simulink model "PV_GFL_864_Average_SM_R1"  (R2026a)
settings: Solver=ode23t  StopTime=0.20  MaxStep=1e-5
InitFcn:
  | run(fullfile(fileparts(get_param(bdroot,'FileName')),'..','scripts','init_pv_gfl_864_average_sm.m'));
undefined symbols (not defined in the file): Control, DiscIntNeverNeededParam, ee, GridTransformer, S1, SM, Ts
libraries: ee_lib x18, nesl_utility x16, fl_lib x10, simulink x1, eeSmAC1C x1
Description:
  | B2 readable SRF-PLL, dq measurement, and P/Q estimation on the validated B1 switching plant.
settings Model: Creator=fakebob2004  LastModifiedBy=fakebob2004

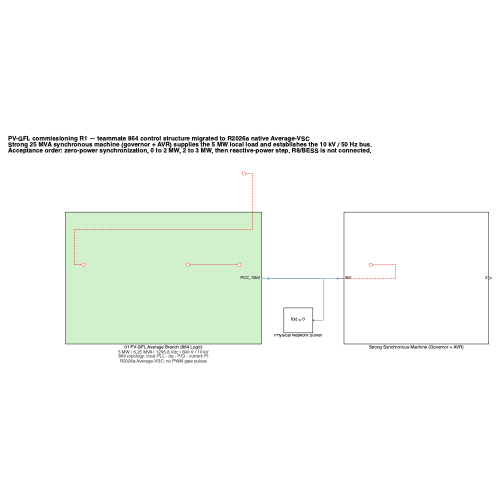
[thumbnail: Simulink's stored preview of the top-level diagram]
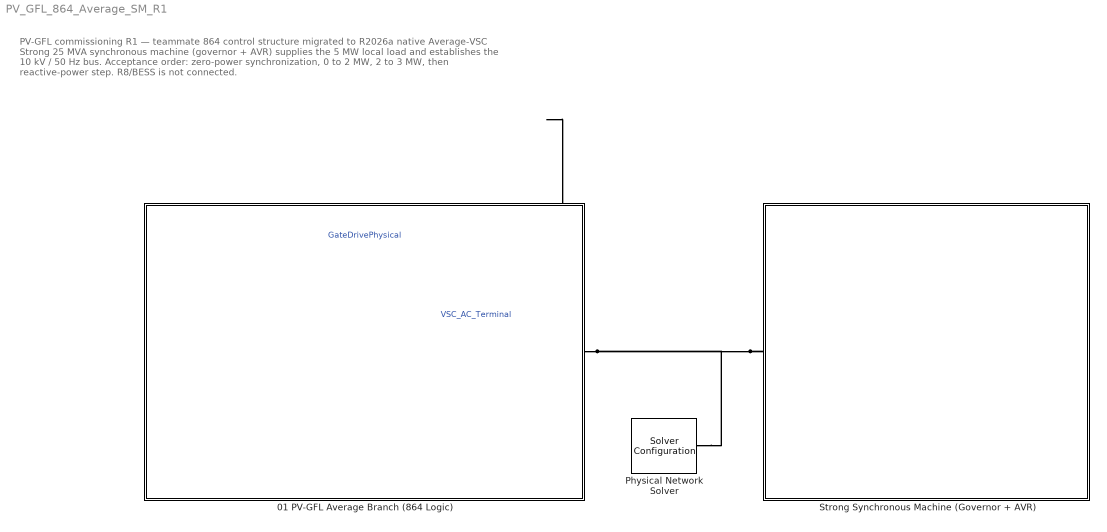
== system PV_GFL_864_Average_SM_R1 ==
  note: PV-GFL commissioning R1 — teammate 864 control structure migrated to R2026a native Average-VSC
      | Strong 25 MVA synchronous machine (governor + AVR) supplies the 5 MW local load and establishes the 10 kV / 50 Hz bus.
      | Acceptance order: zero-power synchronization, 0 to 2 MW, 2 to 3 MW, then reactive-power step. R8/BESS is not connected.
  01 PV-GFL Average Branch (864 Logic) : Subsystem
      settings: AttributesFormatString=|
      | 5 MW / 6.25 MVA | 1295.8 Vdc | 690 V / 10 kV
      | 864 topology: local PLL - dq - P/Q - current PI
      | R2026a Average-VSC; no PWM gate pulses
  Physical Network Solver : nesl_utility/Solver Configuration  PhysicalDomain=network_engine_domain  SubClassName=solver  LeftPortType=input  RightPortType=generic  Tones=[]  Harmonics=[]  SimulateNoise=off  Profile=off  UseLocalSampling=off  EnableSwitchedLinearOptims=on  FrequencyDomain=off  UseCCode=off  RelTol=0.001  AbsTol=0.001  MinStep=1e-09  ToWorkspace=off  RevertToSquareIcSolve=off  NumHomotopyIterations=100  PhasorMode=off  PhasorModeNumHarmonics=1  ConsistencySolver=NEWTON_XTOL_AFTER_FTOL  CanonicalOrdering=CANONICAL  OptimizeIntermediates=OPTIMIZED  IndexReductionMethod=DerivativeReplacement  DoDC=off  ResidualTolerance=1e-09  ConsistencyTolSource=GLOBAL  ConsistencyAbsTol=0.001  ConsistencyRelTol=0.001  ConsistencyTolFactor=0.001  UseLocalSolver=off  LocalSolverChoice=NE_BACKWARD_EULER_ADVANCER  ResolveIndetEquations=on  FunctionEvalNumThread=1  LocalSolverSampleTime=0.001  DoFixedCost=off  MaxNonlinIter=3  MaxModeIter=2  ComputeImpulses=off  ImpulseIterations=2  LinearAlgebra=auto  LinearAlgebraNumThread=0  EquationFormulation=NE_TIME_EF  DelaysMemoryBudget=1024  AutomaticFiltering=on  FilteringTimeConstant=0.001  PartitionStorageMethod=AS_NEEDED  PartitionMemoryBudget=1024  PartitionMethod=ROBUST  MultibodyUseLocalSolver=off  MultibodyLocalSolverChoice=ODE1  MultibodyLocalSolverSampleTime=0.001
  Strong Synchronous Machine (Governor + AVR) : Subsystem  VariantControl=SynchronousMachine
  connections:
  ?  "VSC_AC_Terminal"
  ?  "GateDrivePhysical"
  Strong Synchronous Machine (Governor + AVR)/RConn1 -- 01 PV-GFL Average Branch (864 Logic)/RConn1 -- Physical Network Solver/RConn1

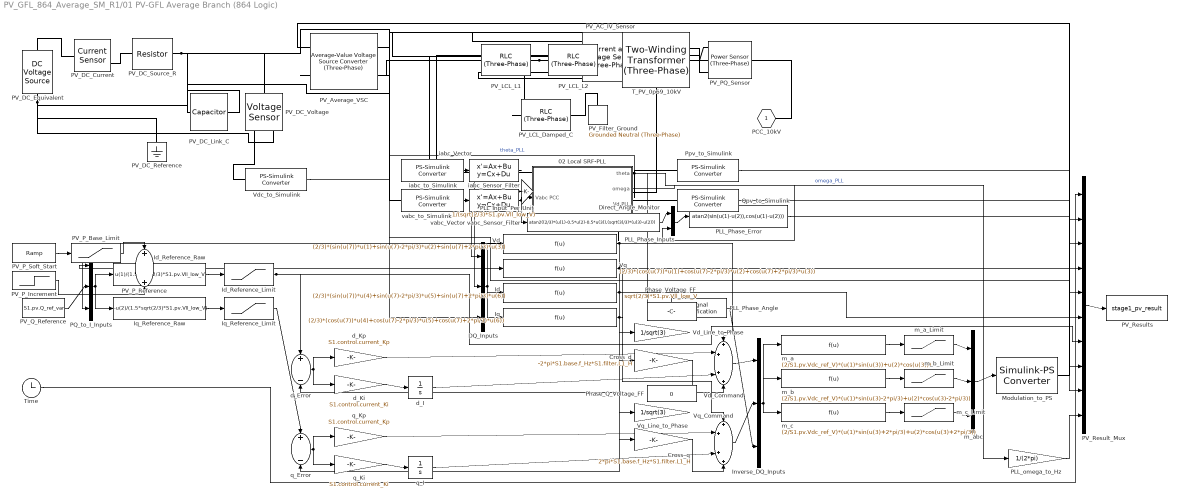
== system PV_GFL_864_Average_SM_R1/01 PV-GFL Average Branch (864 Logic) ==
  02 Local SRF-PLL : Subsystem
  Cross_d : Gain  Gain=-2*pi*S1.base.f_Hz*S1.filter.L1_H
  Cross_q : Gain  Gain=2*pi*S1.base.f_Hz*S1.filter.L1_H
  DQ_Inputs : Mux  Inputs=3
  Direct_Angle_Monitor : Fcn  Expr=atan2((2/3)*(u(1)-0.5*u(2)-0.5*u(3)),(sqrt(3)/3)*(u(3)-u(2)))
  Id : Fcn  Expr=(2/3)*(sin(u(7))*u(4)+sin(u(7)-2*pi/3)*u(5)+sin(u(7)+2*pi/3)*u(6))
  Id_Reference_Limit : Saturate  UpperLimit=S1.control.Ilimit_A  LowerLimit=-S1.control.Ilimit_A
  Id_Reference_Raw : Fcn  Expr=u(1)/(1.5*sqrt(2/3)*S1.pv.Vll_low_V)
  Inverse_DQ_Inputs : Mux  Inputs=3
  Iq : Fcn  Expr=(2/3)*(cos(u(7))*u(4)+cos(u(7)-2*pi/3)*u(5)+cos(u(7)+2*pi/3)*u(6))
  Iq_Reference_Limit : Saturate  UpperLimit=S1.control.Ilimit_A  LowerLimit=-S1.control.Ilimit_A
  Iq_Reference_Raw : Fcn  Expr=-u(2)/(1.5*sqrt(2/3)*S1.pv.Vll_low_V)
  Modulation_to_PS : nesl_utility/Simulink-PS Converter  PhysicalDomain=network_engine_domain  SubClassName=ps_input  LeftPortType=input  RightPortType=output  PseudoPeriodic=off  Frequencies=[]  NoiseDistribution=none  NoiseParameters=[]  Unit=1  AffineConversion=off  FilteringAndDerivatives=zero  SimscapeFilterOrder=1  InputFilterTimeConstant=0.001  UdotUserProvided=0
  PLL_Input_Per_Unit : Gain  Gain=1/(sqrt(2/3)*S1.pv.Vll_low_V)
  PLL_Phase_Angle : SignalSpecification
  PLL_Phase_Error : Fcn  Expr=atan2(sin(u(1)-u(2)),cos(u(1)-u(2)))
  PLL_Phase_Inputs : Mux  Inputs=2
  PLL_omega_to_Hz : Gain  Gain=1/(2*pi)
  PQ_to_I_Inputs : Mux  Inputs=3
  PV_AC_IV_Sensor : ee_lib/Sensors & Transducers/Current and Voltage Sensor (Three-Phase)  port_option=ee.enum.threePhasePort.composite  vMeasurementType=ee.enum.vmeasurement.ll  outputUnit=ee.enum.unit.si  SRated=100e6 A*V  VRated=24e3 V  I_specify=off  I_priority=None  I=[0, 0, 0] A  I_nominal_specify=off  I_nominal_value=1  I_nominal_unit=A  V_specify=off  V_priority=None  V=[0, 0, 0] V  V_nominal_specify=off  V_nominal_value=1  V_nominal_unit=V
  PV_Average_VSC : ee_lib/Semiconductors & Converters/Converters/Average-Value Voltage Source Converter (Three-Phase)  port_option=ee.enum.threePhasePort.composite  enable_block_pulses_input=false  krec=0.001 Ohm  frequency_option=ee.enum.converters.frequency.variable  input_option=ee.enum.converters.inputOption.ModWave  FRated=S1.base.f_Hz Hz  losses_parameterization=ee.enum.converters.losses.fixed  Pfixed=1 W  ks=0.01  kc1=1.7 V  kc2=0.01 Ohm  Ploss_vect=[100, 800, 1870, 3250, 4900] W  Irms_vect=[10, 100, 200, 300, 400] A  Vdc_nom=300 V  thermal_mass=30000 J/K  temperature_specify=off  temperature_priority=High  temperature=298.15 K  temperature_nominal_specify=off  temperature_nominal_value=1  temperature_nominal_unit=K
  PV_DC_Current : fl_lib/Electrical/Electrical Sensors/Current Sensor
  PV_DC_Equivalent : fl_lib/Electrical/Electrical Sources/DC Voltage Source  v0=S1.pv.Vdc_ref_V V
  PV_DC_Link_C : fl_lib/Electrical/Electrical Elements/Capacitor  c=S1.pv.Cdc_F F  r=1e-6 Ohm  g=0 1/Ohm  i_specify=off  i_priority=None  i=0 A  i_nominal_specify=off  i_nominal_value=1  i_nominal_unit=A  v_specify=off  v_priority=None  v=0 V  v_nominal_specify=off  v_nominal_value=1  v_nominal_unit=V  vc_specify=on  vc_priority=High  vc=S1.pv.Vdc_ref_V V  vc_nominal_specify=off  vc_nominal_value=1  vc_nominal_unit=V
  PV_DC_Reference : fl_lib/Electrical/Electrical Elements/Electrical Reference
  PV_DC_Source_R : fl_lib/Electrical/Electrical Elements/Resistor  R=S1.pv.dc_source_R_ohm Ohm  i_specify=off  i_priority=None  i=0 A  i_nominal_specify=off  i_nominal_value=1  i_nominal_unit=A  v_specify=off  v_priority=None  v=0 V  v_nominal_specify=off  v_nominal_value=1  v_nominal_unit=V
  PV_DC_Voltage : fl_lib/Electrical/Electrical Sensors/Voltage Sensor
  PV_Filter_Ground : ee_lib/Connectors & References/Grounded Neutral (Three-Phase)  port_option=ee.enum.threePhasePort.composite
  PV_LCL_Damped_C : ee_lib/Passive/RLC Assemblies/RLC (Three-Phase)  port_option=ee.enum.threePhasePort.composite  component_structure=ee.enum.rlc.structure.SeriesRC  R=S1.filter.Rd_ohm Ohm  L=1e-3 H  C=S1.filter.C_F F  R_parasitic=0 Ohm  G_parasitic=0 1/Ohm  IL_specify=off  IL_priority=High  IL=[0, 0, 0] A  IL_nominal_specify=off  IL_nominal_value=1  IL_nominal_unit=A  VC_specify=off  VC_priority=High  VC=[0, 0, 0] V  VC_nominal_specify=off  VC_nominal_value=1  VC_nominal_unit=V
  PV_LCL_L1 : ee_lib/Passive/RLC Assemblies/RLC (Three-Phase)  port_option=ee.enum.threePhasePort.composite  component_structure=ee.enum.rlc.structure.SeriesRL  R=S1.filter.R1_ohm Ohm  L=S1.filter.L1_H H  C=1e-6 F  R_parasitic=0 Ohm  G_parasitic=0 1/Ohm  IL_specify=off  IL_priority=High  IL=[0, 0, 0] A  IL_nominal_specify=off  IL_nominal_value=1  IL_nominal_unit=A  VC_specify=off  VC_priority=High  VC=[0, 0, 0] V  VC_nominal_specify=off  VC_nominal_value=1  VC_nominal_unit=V
  PV_LCL_L2 : ee_lib/Passive/RLC Assemblies/RLC (Three-Phase)  port_option=ee.enum.threePhasePort.composite  component_structure=ee.enum.rlc.structure.SeriesRL  R=S1.filter.R2_ohm Ohm  L=S1.filter.L2_H H  C=1e-6 F  R_parasitic=0 Ohm  G_parasitic=0 1/Ohm  IL_specify=off  IL_priority=High  IL=[0, 0, 0] A  IL_nominal_specify=off  IL_nominal_value=1  IL_nominal_unit=A  VC_specify=off  VC_priority=High  VC=[0, 0, 0] V  VC_nominal_specify=off  VC_nominal_value=1  VC_nominal_unit=V
  PV_PQ_Sensor : ee_lib/Sensors & Transducers/Power Sensor (Three-Phase)  port_option=ee.enum.threePhasePort.composite  load_type=ee.enum.passive.type_balanced.balanced  f0=60 Hz
  PV_P_Base_Limit : Saturate  UpperLimit=S1.pv.P_initial_W  LowerLimit=0
  PV_P_Increment : Step  Time=S1.pv.P_step_time_s  FinalValue=S1.pv.P_final_W-S1.pv.P_initial_W  SampleTime=0
  PV_P_Reference : Sum
  PV_P_Soft_Start : simulink/Sources/Ramp  slope=S1.pv.P_ramp_W_per_s  start=0  InitialOutput=0
  PV_Q_Reference : Constant  Value=S1.pv.Q_ref_var
  PV_Result_Mux : Mux  Inputs=10
  PV_Results : ToWorkspace  VariableName=stage1_pv_result  SampleTime=-1
  Phase_Q_Voltage_FF : Constant  Value=0
  Phase_Voltage_FF : Constant  Value=sqrt(2/3)*S1.pv.Vll_low_V
  Ppv_to_Simulink : nesl_utility/PS-Simulink Converter  PhysicalDomain=network_engine_domain  SubClassName=ps_output  LeftPortType=input  RightPortType=output  PseudoPeriodic=off  Frequencies=[]  VectorFormat=inherit  Unit=W  AffineConversion=off
  Qpv_to_Simulink : nesl_utility/PS-Simulink Converter  PhysicalDomain=network_engine_domain  SubClassName=ps_output  LeftPortType=input  RightPortType=output  PseudoPeriodic=off  Frequencies=[]  VectorFormat=inherit  Unit=W  AffineConversion=off
  T_PV_0p69_10kV : ee_lib/Passive/Transformers/Two-Winding Transformer (Three-Phase)  SRated=S1.transformer.S_VA A*V  FRated=S1.base.f_Hz Hz  Winding1Connection=ee.enum.windingconnection.delta1  VRated1=S1.pv.Vll_low_V V  Winding2Connection=ee.enum.windingconnection.Yg  VRated2=S1.pv.Vll_high_V V  CoreType=ee.enum.coretype.threelimb  pu_Rw1=S1.transformer.R_pu/2  pu_Rw2=S1.transformer.R_pu/2  leakage_reactance_option=ee.enum.transformer_leakage.include  pu_Xl1=S1.transformer.X_pu/2  pu_Xl2=S1.transformer.X_pu/2  magnetizing_resistance_option=ee.enum.transformer_magnetizingResistance.exclude  pu_Rm=500  magnetizing_reactance_option=ee.enum.transformer_magnetizingReactance.exclude  saturation_option=ee.enum.transformer_saturation.exclude  pu_Xm=500  current_data=[0, .002, 1, 2]  magnetic_flux_data=[0, 1.2, 1.5, 1.51]  pu_X0=0.5  i1_specify=off  i1_priority=None  i1=[0, 0, 0] A  i1_nominal_specify=off  i1_nominal_value=1  i1_nominal_unit=A  i2_specify=off  i2_priority=None  i2=[0, 0, 0] A  i2_nominal_specify=off  i2_nominal_value=1  i2_nominal_unit=A  phi_specify=off  phi_priority=None  phi=[0, 0, 0]  phi_nominal_specify=off  phi_nominal_value=1  phi_nominal_unit=1
  Time : Clock
  Vd : Fcn  Expr=(2/3)*(sin(u(7))*u(1)+sin(u(7)-2*pi/3)*u(2)+sin(u(7)+2*pi/3)*u(3))
  Vd_Command : Sum  Inputs=++++
  Vd_Line_to_Phase : Gain  Gain=1/sqrt(3)
  Vdc_to_Simulink : nesl_utility/PS-Simulink Converter  PhysicalDomain=network_engine_domain  SubClassName=ps_output  LeftPortType=input  RightPortType=output  PseudoPeriodic=off  Frequencies=[]  VectorFormat=inherit  Unit=V  AffineConversion=off
  Vq : Fcn  Expr=(2/3)*(cos(u(7))*u(1)+cos(u(7)-2*pi/3)*u(2)+cos(u(7)+2*pi/3)*u(3))
  Vq_Command : Sum  Inputs=++++
  Vq_Line_to_Phase : Gain  Gain=1/sqrt(3)
  d_Error : Sum  Inputs=+-
  d_I : Integrator
  d_Ki : Gain  Gain=S1.control.current_Ki
  d_Kp : Gain  Gain=S1.control.current_Kp
  iabc_Sensor_Filter : StateSpace  A=-eye(3)/S1.control.sensor_filter_s  B=eye(3)/S1.control.sensor_filter_s  C=eye(3)  D=zeros(3)  InitialCondition=zeros(3,1)
  iabc_Vector : Reshape
  iabc_to_Simulink : nesl_utility/PS-Simulink Converter  PhysicalDomain=network_engine_domain  SubClassName=ps_output  LeftPortType=input  RightPortType=output  PseudoPeriodic=off  Frequencies=[]  VectorFormat=inherit  Unit=A  AffineConversion=off
  m_a : Fcn  Expr=(2/S1.pv.Vdc_ref_V)*(u(1)*sin(u(3))+u(2)*cos(u(3)))
  m_a_Limit : Saturate  UpperLimit=S1.pv.modulation_max  LowerLimit=-S1.pv.modulation_max
  m_abc : Mux  Inputs=3
  m_b : Fcn  Expr=(2/S1.pv.Vdc_ref_V)*(u(1)*sin(u(3)-2*pi/3)+u(2)*cos(u(3)-2*pi/3))
  m_b_Limit : Saturate  UpperLimit=S1.pv.modulation_max  LowerLimit=-S1.pv.modulation_max
  m_c : Fcn  Expr=(2/S1.pv.Vdc_ref_V)*(u(1)*sin(u(3)+2*pi/3)+u(2)*cos(u(3)+2*pi/3))
  m_c_Limit : Saturate  UpperLimit=S1.pv.modulation_max  LowerLimit=-S1.pv.modulation_max
  q_Error : Sum  Inputs=+-
  q_I : Integrator
  q_Ki : Gain  Gain=S1.control.current_Ki
  q_Kp : Gain  Gain=S1.control.current_Kp
  vabc_Sensor_Filter : StateSpace  A=-eye(3)/S1.control.sensor_filter_s  B=eye(3)/S1.control.sensor_filter_s  C=eye(3)  D=zeros(3)  InitialCondition=sqrt(2/3)*S1.pv.Vll_low_V*[sin(pi/6);sin(pi/6-2*pi/3);sin(pi/6+2*pi/3)]
  vabc_Vector : Reshape
  vabc_to_Simulink : nesl_utility/PS-Simulink Converter  PhysicalDomain=network_engine_domain  SubClassName=ps_output  LeftPortType=input  RightPortType=output  PseudoPeriodic=off  Frequencies=[]  VectorFormat=inherit  Unit=V  AffineConversion=off
  PCC_10kV : PMIOPort  Side=Right  ConnectionType=Connection: foundation.electrical.three_phase
  wires:
  PV_Result_Mux/1 -> PV_Results/1
  Vdc_to_Simulink/1 -> PV_Result_Mux/9
  PLL_Phase_Error/1 -> PV_Result_Mux/5
  Qpv_to_Simulink/1 -> PV_Result_Mux/3
  Ppv_to_Simulink/1 -> PV_Result_Mux/2
  Time/1 -> PV_Result_Mux/1
  m_abc/1 -> Modulation_to_PS/1
  m_c_Limit/1 -> m_abc/3
  m_b_Limit/1 -> m_abc/2
  m_a_Limit/1 -> m_abc/1
  m_c/1 -> m_c_Limit/1
  m_b/1 -> m_b_Limit/1
  m_a/1 -> m_a_Limit/1
  Inverse_DQ_Inputs/1 -> m_c/1, m_b/1, m_a/1
  PLL_Phase_Angle/1 -> Inverse_DQ_Inputs/3
  Vq_Command/1 -> Inverse_DQ_Inputs/2
  Vd_Command/1 -> Inverse_DQ_Inputs/1
  Cross_q/1 -> Vq_Command/4
  q_I/1 -> Vq_Command/3
  q_Kp/1 -> Vq_Command/2
  Cross_d/1 -> Vd_Command/4
  d_I/1 -> Vd_Command/3
  d_Kp/1 -> Vd_Command/2
  Vq/1 -> Vq_Line_to_Phase/1, Vq_Command/1
  Iq/1 -> PV_Result_Mux/7, Cross_d/1, q_Error/2
  Iq_Reference_Limit/1 -> q_Error/1
  Id/1 -> PV_Result_Mux/6, Cross_q/1, d_Error/2
  Id_Reference_Limit/1 -> PV_Result_Mux/8, d_Error/1
  q_Ki/1 -> q_I/1
  q_Error/1 -> q_Ki/1, q_Kp/1
  d_Ki/1 -> d_I/1
  d_Error/1 -> d_Ki/1, d_Kp/1
  Iq_Reference_Raw/1 -> Iq_Reference_Limit/1
  Id_Reference_Raw/1 -> Id_Reference_Limit/1
  PQ_to_I_Inputs/1 -> Iq_Reference_Raw/1, Id_Reference_Raw/1
  Vd/1 -> Vd_Line_to_Phase/1, PQ_to_I_Inputs/3, Vd_Command/1
  PV_Q_Reference/1 -> PQ_to_I_Inputs/2
  PV_P_Reference/1 -> PV_Result_Mux/4, PQ_to_I_Inputs/1
  PV_P_Increment/1 -> PV_P_Reference/2
  PV_P_Base_Limit/1 -> PV_P_Reference/1
  PV_P_Soft_Start/1 -> PV_P_Base_Limit/1
  DQ_Inputs/1 -> Iq/1, Id/1, Vq/1, Vd/1
  iabc_Sensor_Filter/1 -> DQ_Inputs/2
  PLL_Phase_Inputs/1 -> PLL_Phase_Error/1
  Direct_Angle_Monitor/1 -> PLL_Phase_Inputs/1
  vabc_Sensor_Filter/1 -> DQ_Inputs/1, Direct_Angle_Monitor/1, PLL_Input_Per_Unit/1, 02 Local SRF-PLL/1(Vabc PCC)
  vabc_Vector/1 -> vabc_Sensor_Filter/1
  iabc_Vector/1 -> iabc_Sensor_Filter/1
  vabc_to_Simulink/1 -> vabc_Vector/1
  iabc_to_Simulink/1 -> iabc_Vector/1
  02 Local SRF-PLL/1(theta) -> PLL_Phase_Inputs/2, DQ_Inputs/3, PLL_Phase_Angle/1  "theta_PLL"
  02 Local SRF-PLL/2(omega) -> PLL_omega_to_Hz/1  "omega_PLL"
  PLL_omega_to_Hz/1 -> PV_Result_Mux/10
  connections:
  Modulation_to_PS/RConn1 -- PV_Average_VSC/LConn1
  PV_DC_Voltage/RConn1 -- Vdc_to_Simulink/LConn1
  PV_PQ_Sensor/LConn3 -- Qpv_to_Simulink/LConn1
  PV_PQ_Sensor/LConn2 -- Ppv_to_Simulink/LConn1
  PV_AC_IV_Sensor/RConn1 -- vabc_to_Simulink/LConn1
  PV_AC_IV_Sensor/RConn2 -- iabc_to_Simulink/LConn1
  PV_PQ_Sensor/RConn1 -- PCC_10kV/RConn1
  T_PV_0p69_10kV/RConn1 -- PV_PQ_Sensor/LConn1
  PV_LCL_Damped_C/RConn1 -- PV_Filter_Ground/LConn1
  PV_LCL_Damped_C/LConn1 -- PV_LCL_L1/RConn1 -- PV_LCL_L2/LConn1
  PV_DC_Reference/LConn1 -- PV_DC_Voltage/RConn2 -- PV_DC_Link_C/RConn1 -- PV_DC_Equivalent/RConn1 -- PV_Average_VSC/RConn2
  PV_DC_Voltage/LConn1 -- PV_DC_Link_C/LConn1 -- PV_DC_Source_R/RConn1 -- PV_Average_VSC/RConn1
  PV_DC_Current/RConn2 -- PV_DC_Source_R/LConn1
  PV_DC_Equivalent/LConn1 -- PV_DC_Current/LConn1
  PV_Average_VSC/LConn2 -- PV_LCL_L1/LConn1
  PV_LCL_L2/RConn1 -- PV_AC_IV_Sensor/LConn1
  PV_AC_IV_Sensor/RConn3 -- T_PV_0p69_10kV/LConn1

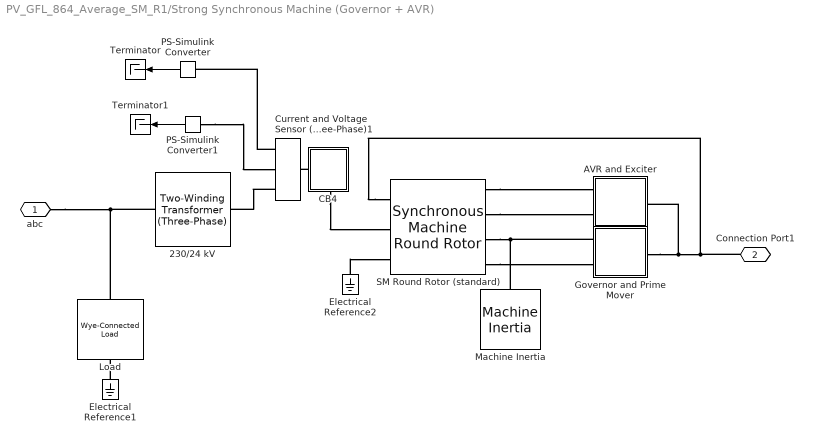
== system PV_GFL_864_Average_SM_R1/Strong Synchronous Machine (Governor + AVR) ==
  " Load" : ee_lib/Passive/RLC Assemblies/Wye-Connected Load  port_option=ee.enum.threePhasePort.composite  parameterization=ee.enum.rlc.parameterization.ratedpower  component_structure=ee.enum.rlc.structure.R  component_structure_PQ=ee.enum.rlc.structure.ParallelRL  R=1 Ohm  L=1e-3 H  C=1e-6 F  VRated=Grid.voltage V  FRated=Grid.frequency Hz  P=SM.P_load W  Qpos=SM.Q_load A*V  Qneg=-1e2 A*V  R_parasitic=0 Ohm  G_parasitic=0 1/Ohm  R_parasitic_PQ=0 Ohm  G_parasitic_PQ=0 1/Ohm  Vmag0=4.16e3 V  Vang0=0 deg  Freq0=60 Hz  IL_specify=off  IL_priority=High  IL=[0, 0, 0] A  IL_nominal_specify=off  IL_nominal_value=1  IL_nominal_unit=A  VC_specify=off  VC_priority=High  VC=[0, 0, 0] V  VC_nominal_specify=off  VC_nominal_value=1  VC_nominal_unit=V
  230/24 kV : ee_lib/Passive/Transformers/Two-Winding Transformer (Three-Phase)  SRated=SM.MVA V*A  FRated=Grid.frequency Hz  Winding1Connection=ee.enum.windingconnection.delta1  VRated1=Grid.voltage V  Winding2Connection=ee.enum.windingconnection.delta11  VRated2=SM.Voltage V  CoreType=ee.enum.coretype.fivelimb  pu_Rw1=GridTransformer.winding_resistance/2  pu_Rw2=GridTransformer.winding_resistance/2  leakage_reactance_option=ee.enum.transformer_leakage.include  pu_Xl1=GridTransformer.winding_lekage_reactance/2  pu_Xl2=GridTransformer.winding_lekage_reactance/2  magnetizing_resistance_option=ee.enum.transformer_magnetizingResistance.exclude  pu_Rm=500  magnetizing_reactance_option=ee.enum.transformer_magnetizingReactance.include  saturation_option=ee.enum.transformer_saturation.exclude  pu_Xm=500  current_data=[0, .002, 1, 2]  magnetic_flux_data=[0, 1.2, 1.5, 1.51]  pu_X0=0.0586/2  i1_specify=off  i1_priority=None  i1=[ 0 0 0 ] A  i1_nominal_specify=off  i1_nominal_value=1  i1_nominal_unit=A  i2_specify=off  i2_priority=None  i2=[ 0 0 0 ] A  i2_nominal_specify=off  i2_nominal_value=1  i2_nominal_unit=A  phi_specify=off  phi_priority=None  phi=[ 0 0 0 ]  phi_nominal_specify=off  phi_nominal_value=1  phi_nominal_unit=1
  AVR and Exciter : Subsystem
  CB4 : Subsystem
      settings: PortSchema="{\"entries\":[{\"content\":{\"sides\":[{\"content\":{\"connectorIds\":[\"LConn1\"]},\"type\":\"ConnectorPlacement.EquallySpacedRectSide\",\"uuid\":\"24022911-97b6-486c-a625-f0780a134feb\"},{\"content\":{\"connectorIds\":[],\"side\":\"RIGHT\"},\"type\":\"ConnectorPlacement.EquallySpacedRectSide\",\"uuid\":\"1242aa8b-343b-4af2-8b96-dfa58505a53d\"},{\"content\":{\"connectorIds\":[],\"side\":\"TOP\"},\"type\":\"ConnectorPlacement.EquallySpacedRectSide\",\"uuid\":\"e73be2e9-5300-480f-914f-665ff518f6ad\"},{\"content\":{\"connectorIds\":[\"RConn1\"],\"side\":\"BOTTOM\"},\"type\":\"ConnectorPlacement.EquallySpacedRectSide\",\"uuid\":\"6525202c-c4e7-4c96-9421-427b801d0594\"}]},\"type\":\"ConnectorPlacement.EquallySpacedConnector\",\"uuid\":\"b455682c-e951-4ef6-bff8-cd3f50b315f1\"}],\"packageUris\":[\"http://schema.mathworks.com/mf0/Connector/R2020b\"],\"version\":\"1.0\"}"
      mask Display: image('$imagefile'); % Use "Edit Image" on toolstrip to change.
  Current and Voltage Sensor (Three-Phase)1 : ee_lib/Sensors & Transducers/Current and Voltage Sensor (Three-Phase)  port_option=ee.enum.threePhasePort.composite  vMeasurementType=ee.enum.vmeasurement.ll  outputUnit=ee.enum.unit.pu  SRated=100e6 A*V  VRated=4.16e3 V  I_specify=off  I_priority=None  I=[0, 0, 0] A  I_nominal_specify=off  I_nominal_value=1  I_nominal_unit=A  V_specify=off  V_priority=None  V=[0, 0, 0] V  V_nominal_specify=off  V_nominal_value=1  V_nominal_unit=V
  Electrical Reference1 : fl_lib/Electrical/Electrical Elements/Electrical Reference
  Electrical Reference2 : fl_lib/Electrical/Electrical Elements/Electrical Reference
  "Governor and Prime Mover " : Subsystem  mask(Governor and Prime Mover){pu_speed_reference=SM.speed_reference, droop_percentage=SM.droop_p, pu_load_reference_setpoint=SM.load_reference_set_point, T_G=SM.governor_time_constant, T_CH=SM.time_constsnt_steamchest, base_torque=SM.Base_Torque_SM, pu_torque0=SM.initial_torque}
      mask prompts: pu_speed_reference "Speed reference, (pu)"; droop_percentage "Percentage droop, (%)"; pu_load_reference_setpoint "Load reference setpoint, (pu)"; T_G "Time constant of governor, (s)"; T_CH "Time constant of main inlet volumes and steam chest, (s)"; base_torque "Base torque, (N*m)"; pu_torque0 "Initial torque, (pu)"
      mask help:
      | Implements a synchronous machine governor and prime mover. The prime mover is a non-reheat steam turbine.
      |
      | The input to the block is a per-unit synchronous machine measurement vector.
      |
      | R and C are mechanical rotational ports.
  Machine Inertia : ee_lib/Electromechanical/Mechanical/Machine Inertia  SRated=SM.MVA V*A  FRated=Grid.frequency Hz  nPolePairs=SM.polepairs  inertia_option=2  J=27548 kg*m^2  H=SM.inertia s  damper_option=2  D=39.0509 N*m/(rad/s)  pu_D=SM.damping  initialization_option=2  fMechanical0=60 Hz  fElectrical0=Grid.frequency Hz
  PS-Simulink Converter : nesl_utility/PS-Simulink Converter  PhysicalDomain=network_engine_domain  SubClassName=ps_output  LeftPortType=input  RightPortType=output  PseudoPeriodic=off  Frequencies=[]  VectorFormat=inherit  Unit=inherit  AffineConversion=off
  PS-Simulink Converter1 : nesl_utility/PS-Simulink Converter  PhysicalDomain=network_engine_domain  SubClassName=ps_output  LeftPortType=input  RightPortType=output  PseudoPeriodic=off  Frequencies=[]  VectorFormat=inherit  Unit=inherit  AffineConversion=off
  SM Round Rotor (standard) : ee_lib/Electromechanical/Synchronous/Synchronous Machine Round Rotor  port_option=ee.enum.threePhasePort.composite  SRated=SM.MVA V*A  VRated=SM.Voltage V  FRated=Grid.frequency Hz  nPolePairs=SM.polepairs  param_option=ee.enum.sm.parameterization.standard  fieldCircuitParameterization_option=2  baseEfd=92.95 V  baseIfd=SM.field_current A  zero_sequence=ee.enum.park.zerosequence.include  axes_param=ee.enum.rotorangle.qaxis  Ladu=1.66  Laqu=1.61  L0=0.15  Ll=0.15  Ra=SM.stator_resistance  Lfd=0.165  Rfd=0.0006  L1d=0.1713  R1d=0.0284  L1q=0.7252  R1q=0.00619  L2q=0.125  R2q=0.02368  Xl=SM.lekage_reactance  Xd=SM.xd  Xq=SM.xq  X0=0.15  Xdd=SM.xd_  Xqd=SM.xq_  Xddd=SM.xd_dash  Xqdd=SM.xq_dash  d_option=1  Td0d=SM.Tdo_ s  Tdd=1.3260 s  Td0dd=SM.Tdo_dash s  Tddd=0.0230 s  q_option=1  Tq0d=SM.Tqo_ s  Tqd=0.3693 s  Tq0dd=SM.Tqo_dash s  Tqdd=0.0269 s  saturation_option=0  saturation_ifd=[0.00, 0.48, 0.76, 1.38, 1.79]  saturation_Vag=[0.00, 0.80, 1.08, 1.31, 1.40]  initialization_option=2  source_type=ee.enum.sm.load_flow_source_type.Swing  Vmag0=SM.Voltage V  Vang0=0 deg  Pt0=SM.initial_Pe V*A  Qt0=SM.initial_Qe V*A  minimum_pu=0.95  phase_search_range=[-inf, inf] deg  gmin=1e-6 S  connection_option=int32(ee.enum.Connection.wye)  num_q_dampers=2  rotor_offset=-pi / 2 rad  pu_psid_specify=on  pu_psid_priority=High  pu_psid=0  pu_psid_nominal_specify=off  pu_psid_nominal_value=1  pu_psid_nominal_unit=1  pu_psiq_specify=on  pu_psiq_priority=High  pu_psiq=0  pu_psiq_nominal_specify=off  pu_psiq_nominal_value=1  pu_psiq_nominal_unit=1  pu_psifd_specify=on  pu_psifd_priority=High  pu_psifd=0  pu_psifd_nominal_specify=off  pu_psifd_nominal_value=1  pu_psifd_nominal_unit=1  pu_psi1d_specify=on  pu_psi1d_priority=High  pu_psi1d=0  pu_psi1d_nominal_specify=off  pu_psi1d_nominal_value=1  pu_psi1d_nominal_unit=1  pu_psi1q_specify=on  pu_psi1q_priority=High  pu_psi1q=0  pu_psi1q_nominal_specify=off  pu_psi1q_nominal_value=1  pu_psi1q_nominal_unit=1  pu_psi2q_specify=on  pu_psi2q_priority=High  pu_psi2q=0  pu_psi2q_nominal_specify=off  pu_psi2q_nominal_value=1  pu_psi2q_nominal_unit=1  angular_position_diff_specify=on  angular_position_diff_priority=High  angular_position_diff=0 deg  angular_position_diff_nominal_specify=off  angular_position_diff_nominal_value=1  angular_position_diff_nominal_unit=deg  Tmeas=298.15 K  alpha=3.93e-3 1/K  stator_thermal_mass=100 J/K  rotor_thermal_mass=200 J/K  temperatureA_specify=off  temperatureA_priority=High  temperatureA=25 degC  temperatureA_nominal_specify=off  temperatureA_nominal_value=1  temperatureA_nominal_unit=degC  temperatureB_specify=off  temperatureB_priority=High  temperatureB=25 degC  temperatureB_nominal_specify=off  temperatureB_nominal_value=1  temperatureB_nominal_unit=degC  temperatureC_specify=off  temperatureC_priority=High  temperatureC=25 degC  temperatureC_nominal_specify=off  temperatureC_nominal_value=1  temperatureC_nominal_unit=degC  temperatureR_specify=off  temperatureR_priority=High  temperatureR=25 degC  temperatureR_nominal_specify=off  temperatureR_nominal_value=1  temperatureR_nominal_unit=degC
  Terminator : Terminator
  Terminator1 : Terminator
  abc : PMIOPort  Side=Right
  Connection Port1 : PMIOPort  Port=2  Side=Left
  wires:
  PS-Simulink Converter1/1 -> Terminator1/1
  PS-Simulink Converter/1 -> Terminator/1
  connections:
  Electrical Reference2/LConn1 -- SM Round Rotor (standard)/RConn3
  CB4/RConn1 -- SM Round Rotor (standard)/RConn2
  PS-Simulink Converter1/LConn1 -- Current and Voltage Sensor (Three-Phase)1/RConn2
  Current and Voltage Sensor (Three-Phase)1/RConn3 -- 230/24 kV/RConn1
  SM Round Rotor (standard)/LConn2 -- AVR and Exciter/RConn2
  Electrical Reference1/LConn1 -- " Load"/RConn1
  CB4/LConn1 -- Current and Voltage Sensor (Three-Phase)1/LConn1
  SM Round Rotor (standard)/LConn1 -- AVR and Exciter/RConn1
  Current and Voltage Sensor (Three-Phase)1/RConn1 -- PS-Simulink Converter/LConn1
  SM Round Rotor (standard)/LConn4 -- "Governor and Prime Mover "/RConn2
  "Governor and Prime Mover "/RConn1 -- Machine Inertia/LConn1 -- SM Round Rotor (standard)/LConn3
  SM Round Rotor (standard)/RConn1 -- Connection Port1/RConn1 -- AVR and Exciter/LConn1 -- "Governor and Prime Mover "/LConn1
  230/24 kV/LConn1 -- abc/RConn1 -- " Load"/LConn1

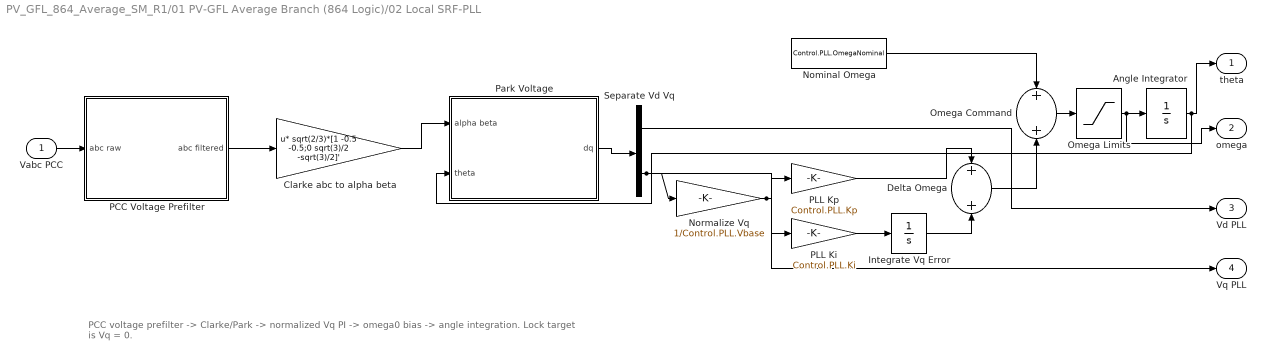
== system PV_GFL_864_Average_SM_R1/01 PV-GFL Average Branch (864 Logic)/02 Local SRF-PLL ==
  note: PCC voltage prefilter -> Clarke/Park -> normalized Vq PI -> omega0 bias -> angle integration. Lock target is Vq = 0.
  Vabc PCC : Inport
  Angle Integrator : Integrator  InitialCondition=Control.PLL.Theta0
  Clarke abc to alpha beta : Gain  Gain=sqrt(2/3)*[1 -0.5 -0.5;0 sqrt(3)/2 -sqrt(3)/2]'  Multiplication=Matrix(u*K)
  Delta Omega : Sum
  Integrate Vq Error : Integrator
  Nominal Omega : Constant  Value=Control.PLL.OmegaNominal
  Normalize Vq : Gain  Gain=1/Control.PLL.Vbase
  Omega Command : Sum
  Omega Limits : Saturate  UpperLimit=Control.PLL.OmegaMax  LowerLimit=Control.PLL.OmegaMin
  PCC Voltage Prefilter : Subsystem
  PLL Ki : Gain  Gain=Control.PLL.Ki
  PLL Kp : Gain  Gain=Control.PLL.Kp
  Park Voltage : Subsystem
  Separate Vd Vq : Demux  Outputs=2
  theta : Outport
  omega : Outport  Port=2
  Vd PLL : Outport  Port=3
  Vq PLL : Outport  Port=4
  wires:
  Separate Vd Vq/1 -> Vd PLL/1
  Omega Limits/1 -> omega/1, Angle Integrator/1
  Omega Command/1 -> Omega Limits/1
  Delta Omega/1 -> Omega Command/2
  Nominal Omega/1 -> Omega Command/1
  Integrate Vq Error/1 -> Delta Omega/2
  PLL Kp/1 -> Delta Omega/1
  PLL Ki/1 -> Integrate Vq Error/1
  Normalize Vq/1 -> PLL Ki/1, PLL Kp/1
  Separate Vd Vq/2 -> Vq PLL/1, Normalize Vq/1
  Park Voltage/1(dq) -> Separate Vd Vq/1
  Angle Integrator/1 -> theta/1, Park Voltage/2(theta)
  Clarke abc to alpha beta/1 -> Park Voltage/1(alpha beta)
  PCC Voltage Prefilter/1(abc filtered) -> Clarke abc to alpha beta/1
  Vabc PCC/1 -> PCC Voltage Prefilter/1(abc raw)

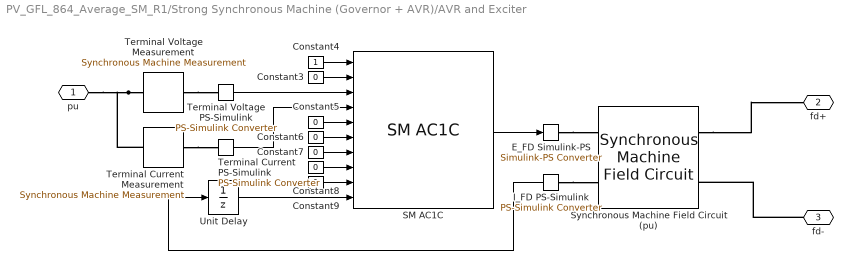
== system PV_GFL_864_Average_SM_R1/Strong Synchronous Machine (Governor + AVR)/AVR and Exciter ==
  Constant{3,5..9} (6 alike) : Constant  Value=0
  Constant4 : Constant
  "E_FD Simulink-PS " : nesl_utility/Simulink-PS Converter  PhysicalDomain=network_engine_domain  SubClassName=ps_input  LeftPortType=input  RightPortType=output  PseudoPeriodic=off  Frequencies=[]  NoiseDistribution=none  NoiseParameters=[]  Unit=1  AffineConversion=off  FilteringAndDerivatives=zero  SimscapeFilterOrder=1  InputFilterTimeConstant=.001  UdotUserProvided=0
  I_FD PS-Simulink : nesl_utility/PS-Simulink Converter  PhysicalDomain=network_engine_domain  SubClassName=ps_output  LeftPortType=input  RightPortType=output  PseudoPeriodic=off  Frequencies=[]  VectorFormat=1-D array  Unit=1  AffineConversion=off
  SM AC1C : eeSmAC1C/SM AC1C  E_FD0=1  Ts=-1  R_C=0  X_C=0  T_R=0  K_A=600  T_A=0.01  T_B=0  T_C=0  K_F=0.35  T_F=0.5  V_Amax=14.5  V_Amin=-14.5  E_FEmax=6.03  E_FEmin=-5.43  oelInputLocation=Unused  uelInputLocation=Unused  sclInputLocation=Unused  K_E=1  T_E=0.08  K_C=0.2  K_D=0.38  E_1=4.18  S_E_E1=0.1  E_2=3.14  S_E_E2=0.03  V_FEmax=99  V_Emin=0
  Synchronous Machine Field Circuit (pu) : ee_lib/Electromechanical/Synchronous/Synchronous Machine Field Circuit  unit_option=ee.enum.unit.pu  SRated=SM.MVA V*A  FRated=60 Hz  fieldCircuitParameterization_option=2  baseEfd=92.95 V  baseIfd=1300 A  parameterization_option=2  Ladu=1.66  Rfd=0.0006  Xl=SM.lekage_reactance  Xd=SM.xd  Xdd=SM.xd_  Xddd=SM.xd_dash  d_option=ee.enum.circuit.open  Td0d=SM.Tdo_ s  Tdd=1.3260 s  Td0dd=SM.Tdo_dash s  Tddd=0.0230 s
  Terminal Current Measurement : ee_lib/Electromechanical/Synchronous/Synchronous Machine Measurement  output_idx=15
  Terminal Current PS-Simulink : nesl_utility/PS-Simulink Converter  PhysicalDomain=network_engine_domain  SubClassName=ps_output  LeftPortType=input  RightPortType=output  PseudoPeriodic=off  Frequencies=[]  VectorFormat=1-D array  Unit=1  AffineConversion=off
  Terminal Voltage Measurement : ee_lib/Electromechanical/Synchronous/Synchronous Machine Measurement  output_idx=14
  Terminal Voltage PS-Simulink : nesl_utility/PS-Simulink Converter  PhysicalDomain=network_engine_domain  SubClassName=ps_output  LeftPortType=input  RightPortType=output  PseudoPeriodic=off  Frequencies=[]  VectorFormat=1-D array  Unit=1  AffineConversion=off
  Unit Delay : UnitDelay  InitialCondition=1.32943  SampleTime=-1
  pu : PMIOPort  Side=Left
  fd+ : PMIOPort  Port=2  Side=Right
  fd- : PMIOPort  Port=3  Side=Right
  wires:
  I_FD PS-Simulink/1 -> Unit Delay/1
  Terminal Voltage PS-Simulink/1 -> SM AC1C/3
  Constant3/1 -> SM AC1C/2
  Constant4/1 -> SM AC1C/1
  Constant5/1 -> SM AC1C/5
  Constant6/1 -> SM AC1C/6
  Constant7/1 -> SM AC1C/7
  Constant8/1 -> SM AC1C/8
  Constant9/1 -> SM AC1C/9
  Unit Delay/1 -> SM AC1C/10
  SM AC1C/1 -> "E_FD Simulink-PS "/1
  Terminal Current PS-Simulink/1 -> SM AC1C/4
  connections:
  "E_FD Simulink-PS "/RConn1 -- Synchronous Machine Field Circuit (pu)/LConn1
  I_FD PS-Simulink/LConn1 -- Synchronous Machine Field Circuit (pu)/LConn2
  fd-/RConn1 -- Synchronous Machine Field Circuit (pu)/RConn2
  Synchronous Machine Field Circuit (pu)/RConn1 -- fd+/RConn1
  Terminal Voltage Measurement/LConn1 -- Terminal Current Measurement/LConn1 -- pu/RConn1
  Terminal Voltage Measurement/RConn1 -- Terminal Voltage PS-Simulink/LConn1
  Terminal Current Measurement/RConn1 -- Terminal Current PS-Simulink/LConn1

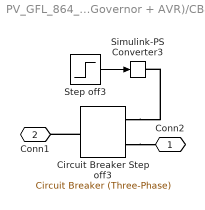
== system PV_GFL_864_Average_SM_R1/Strong Synchronous Machine (Governor + AVR)/CB4 ==
  Circuit Breaker Step off3 : ee_lib/Switches & Breakers/Circuit Breaker (Three-Phase)  port_option=ee.enum.threePhasePort.composite  control_port_option=ee.enum.controlport.ps  R_closed=0.001 Ohm  G_open=1e-4 1/Ohm  threshold=0.5 V  breaker_behavior=ee.enum.switches.breakerBehavior.zeroCrossingEnable  i_th=1e-8 A
  Simulink-PS Converter3 : nesl_utility/Simulink-PS Converter  PhysicalDomain=network_engine_domain  SubClassName=ps_input  LeftPortType=input  RightPortType=output  PseudoPeriodic=off  Frequencies=[]  NoiseDistribution=none  NoiseParameters=[]  Unit=1  AffineConversion=off  FilteringAndDerivatives=zero  SimscapeFilterOrder=1  InputFilterTimeConstant=0.001  UdotUserProvided=1
  Step off3 : Step  Time=0  FinalValue=0  SampleTime=Ts
  Conn2 : PMIOPort  Side=Left
  Conn1 : PMIOPort  Port=2  Side=Right
  wires:
  Step off3/1 -> Simulink-PS Converter3/1
  connections:
  Circuit Breaker Step off3/RConn1 -- Conn1/RConn1
  Circuit Breaker Step off3/LConn1 -- Simulink-PS Converter3/RConn1
  Circuit Breaker Step off3/LConn2 -- Conn2/RConn1

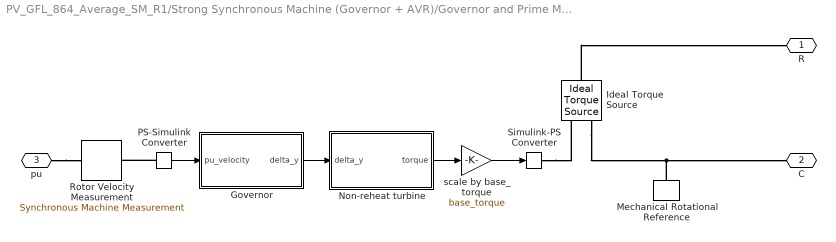
== system PV_GFL_864_Average_SM_R1/Strong Synchronous Machine (Governor + AVR)/Governor and Prime Mover  ==
  Governor : Subsystem
  Ideal Torque Source : fl_lib/Mechanical/Mechanical Sources/Ideal Torque Source
  Mechanical Rotational Reference : fl_lib/Mechanical/Rotational Elements/Mechanical Rotational Reference
  Non-reheat turbine : Subsystem
  PS-Simulink Converter : nesl_utility/PS-Simulink Converter  PhysicalDomain=network_engine_domain  SubClassName=ps_output  LeftPortType=input  RightPortType=output  PseudoPeriodic=off  Frequencies=[]  VectorFormat=1-D array  Unit=1  AffineConversion=off
  Rotor Velocity Measurement : ee_lib/Electromechanical/Synchronous/Synchronous Machine Measurement  output_idx=4
  Simulink-PS Converter : nesl_utility/Simulink-PS Converter  PhysicalDomain=network_engine_domain  SubClassName=ps_input  LeftPortType=input  RightPortType=output  PseudoPeriodic=off  Frequencies=[]  NoiseDistribution=none  NoiseParameters=[]  Unit=1  AffineConversion=off  FilteringAndDerivatives=zero  SimscapeFilterOrder=1  InputFilterTimeConstant=0.001  UdotUserProvided=1
  scale by base_torque : Gain  Gain=base_torque
  R : PMIOPort  Side=Right
  C : PMIOPort  Port=2  Side=Right
  pu : PMIOPort  Port=3  Side=Left
  wires:
  scale by base_torque/1 -> Simulink-PS Converter/1
  Non-reheat turbine/1(torque) -> scale by base_torque/1
  Governor/1(delta_y) -> Non-reheat turbine/1(delta_y)
  PS-Simulink Converter/1 -> Governor/1(pu_velocity)
  connections:
  Simulink-PS Converter/RConn1 -- Ideal Torque Source/RConn1
  PS-Simulink Converter/LConn1 -- Rotor Velocity Measurement/RConn1
  pu/RConn1 -- Rotor Velocity Measurement/LConn1
  Ideal Torque Source/LConn1 -- R/RConn1
  Mechanical Rotational Reference/LConn1 -- Ideal Torque Source/RConn2 -- C/RConn1

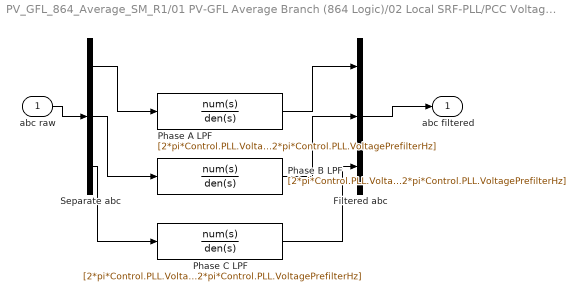
== system PV_GFL_864_Average_SM_R1/01 PV-GFL Average Branch (864 Logic)/02 Local SRF-PLL/PCC Voltage Prefilter ==
  abc raw : Inport
  Filtered abc : Mux  Inputs=3
  Phase A LPF : TransferFcn  Numerator=[2*pi*Control.PLL.VoltagePrefilterHz]  Denominator=[1 2*pi*Control.PLL.VoltagePrefilterHz]
  Phase B LPF : TransferFcn  Numerator=[2*pi*Control.PLL.VoltagePrefilterHz]  Denominator=[1 2*pi*Control.PLL.VoltagePrefilterHz]
  Phase C LPF : TransferFcn  Numerator=[2*pi*Control.PLL.VoltagePrefilterHz]  Denominator=[1 2*pi*Control.PLL.VoltagePrefilterHz]
  Separate abc : Demux  Outputs=3
  abc filtered : Outport
  wires:
  Filtered abc/1 -> abc filtered/1
  abc raw/1 -> Separate abc/1
  Phase C LPF/1 -> Filtered abc/3
  Separate abc/3 -> Phase C LPF/1
  Phase B LPF/1 -> Filtered abc/2
  Separate abc/2 -> Phase B LPF/1
  Phase A LPF/1 -> Filtered abc/1
  Separate abc/1 -> Phase A LPF/1

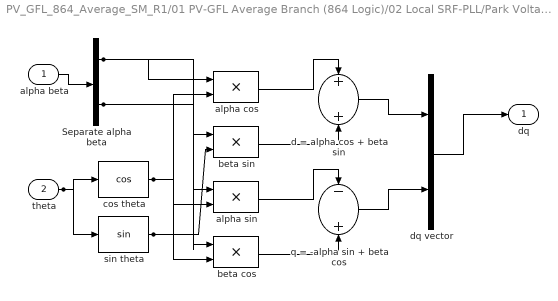
== system PV_GFL_864_Average_SM_R1/01 PV-GFL Average Branch (864 Logic)/02 Local SRF-PLL/Park Voltage ==
  alpha beta : Inport
  theta : Inport  Port=2
  Separate alpha beta : Demux  Outputs=2
  alpha cos : Product
  alpha sin : Product
  beta cos : Product
  beta sin : Product
  cos theta : Trigonometry  Operator=cos
  d = alpha cos + beta sin : Sum
  dq vector : Mux  Inputs=2
  q = -alpha sin + beta cos : Sum  Inputs=-+
  sin theta : Trigonometry
  dq : Outport
  wires:
  dq vector/1 -> dq/1
  q = -alpha sin + beta cos/1 -> dq vector/2
  d = alpha cos + beta sin/1 -> dq vector/1
  beta cos/1 -> q = -alpha sin + beta cos/2
  alpha sin/1 -> q = -alpha sin + beta cos/1
  beta sin/1 -> d = alpha cos + beta sin/2
  alpha cos/1 -> d = alpha cos + beta sin/1
  sin theta/1 -> alpha sin/2, beta sin/2
  Separate alpha beta/2 -> beta cos/1, beta sin/1
  cos theta/1 -> beta cos/2, alpha cos/2
  Separate alpha beta/1 -> alpha sin/1, alpha cos/1
  theta/1 -> sin theta/1, cos theta/1
  alpha beta/1 -> Separate alpha beta/1

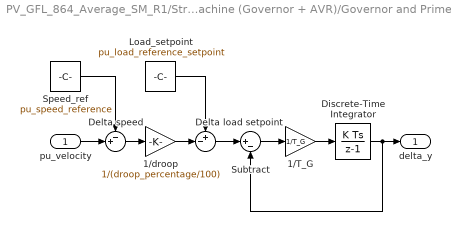
== system PV_GFL_864_Average_SM_R1/Strong Synchronous Machine (Governor + AVR)/Governor and Prime Mover /Governor ==
  pu_velocity : Inport
  1/T_G : Gain  Gain=1/T_G
  1/droop : Gain  Gain=1/(droop_percentage/100)
  Delta load setpoint : Sum  Inputs=+-|
  Delta speed : Sum  Inputs=-+|
  Discrete-Time Integrator : DiscreteIntegrator  InitialCondition=pu_torque0  SampleTime=Ts  ICPrevOutput=DiscIntNeverNeededParam  ICPrevScaledInput=DiscIntNeverNeededParam
  Load_setpoint : Constant  Value=pu_load_reference_setpoint  SampleTime=Ts
  Speed_ref : Constant  Value=pu_speed_reference  SampleTime=Ts
  Subtract : Sum  Inputs=|+-
  delta_y : Outport  VectorParamsAs1DForOutWhenUnconnected=off
  wires:
  Discrete-Time Integrator/1 -> Subtract/2, delta_y/1
  1/T_G/1 -> Discrete-Time Integrator/1
  Subtract/1 -> 1/T_G/1
  Delta load setpoint/1 -> Subtract/1
  1/droop/1 -> Delta load setpoint/2
  pu_velocity/1 -> Delta speed/2
  Load_setpoint/1 -> Delta load setpoint/1
  Delta speed/1 -> 1/droop/1
  Speed_ref/1 -> Delta speed/1

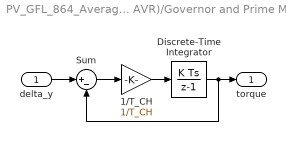
== system PV_GFL_864_Average_SM_R1/Strong Synchronous Machine (Governor + AVR)/Governor and Prime Mover /Non-reheat turbine ==
  delta_y : Inport
  1/T_CH : Gain  Gain=1/T_CH
  Discrete-Time Integrator : DiscreteIntegrator  InitialCondition=pu_torque0  SampleTime=Ts  ICPrevOutput=DiscIntNeverNeededParam  ICPrevScaledInput=DiscIntNeverNeededParam
  Sum : Sum  Inputs=|+-
  torque : Outport  VectorParamsAs1DForOutWhenUnconnected=off
  wires:
  Discrete-Time Integrator/1 -> torque/1, Sum/2
  1/T_CH/1 -> Discrete-Time Integrator/1
  Sum/1 -> 1/T_CH/1
  delta_y/1 -> Sum/1
